simulink model "BFN_00_zfull_system"  (R2019b)
settings: Solver=VariableStepAuto  StartTime=0.0  StopTime=100  RelTol=1e-8
undefined symbols (not defined in the file): agh, Cd, dgh, Eearth, Esun, Gyro_freq, Gyro_noise_b, Gyro_noise_n, IFEHS_noise, Jsc, m_disturb, Magn_noise, q0, Surf_areas, Surf_dist, Surf_normals, Surf_reflectivity, targets_inertial, Tmax, today_mjd2000, w0
libraries: simulink x8, dspsrcs4 x2, vrlib x1
settings Model: Creator=Nicola  LastModifiedBy=Nicola

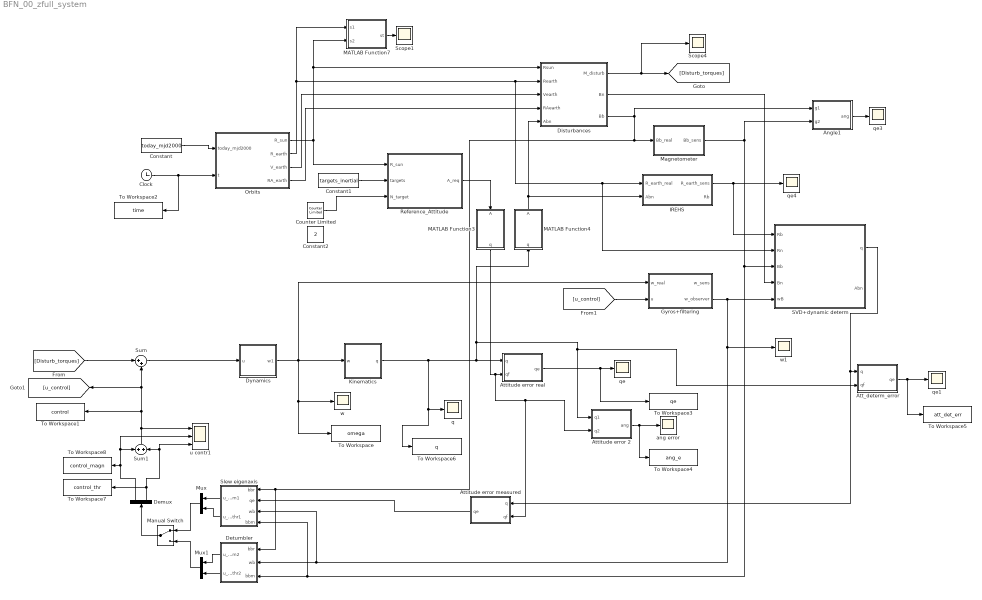
== system BFN_00_zfull_system ==
  Angle1 : MATLAB Function  TreatAsAtomicUnit=on
  Att_determ_error : MATLAB Function  TreatAsAtomicUnit=on
  Attitude error 2 : MATLAB Function  TreatAsAtomicUnit=on
  Attitude error measured : MATLAB Function  TreatAsAtomicUnit=on
  Attitude error real : MATLAB Function  TreatAsAtomicUnit=on
  Clock : Clock
  Constant : Constant  Value=today_mjd2000
  Constant1 : Constant  Value=targets_inertial
  Constant2 : Constant  Value=2
  Counter Limited : simulink/Sources/Counter Limited  uplimit=2  tsamp=6000*3
  Demux : Demux  Outputs=2
  Detumbler : Subsystem
  Disturbances : Subsystem
  Dynamics : Subsystem
  Gyros+filtering : Subsystem
  IREHS : Subsystem
  Kinematics : Subsystem
  MATLAB Function3 : MATLAB Function  TreatAsAtomicUnit=on
  MATLAB Function4 : MATLAB Function  TreatAsAtomicUnit=on
  MATLAB Function7 : MATLAB Function  TreatAsAtomicUnit=on
  Magnetometer : Subsystem
  Manual Switch : ManualSwitch
  Mux : Mux  Inputs=2
  Mux1 : Mux  Inputs=2
  Orbits : MATLAB Function  TreatAsAtomicUnit=on
  Reference_Attitude : MATLAB Function  TreatAsAtomicUnit=on
  SVD+dynamic determ : Subsystem
  Scope1 : Scope
  Scope4 : Scope
  Slew eigenaxis : Subsystem
  Sum : Sum  Inputs=|++
  Sum1 : Sum
  To Workspace : ToWorkspace  VariableName=omega  SampleTime=-1
      settings: Save2DSignal=2-D array (concatenate along first dimension)
  To Workspace1 : ToWorkspace  VariableName=control  SampleTime=-1
      settings: Save2DSignal=2-D array (concatenate along first dimension)
  To Workspace2 : ToWorkspace  VariableName=time  SampleTime=-1
      settings: Save2DSignal=2-D array (concatenate along first dimension)
  To Workspace3 : ToWorkspace  VariableName=qe  SampleTime=-1
      settings: Save2DSignal=2-D array (concatenate along first dimension)
  To Workspace4 : ToWorkspace  VariableName=ang_e  SampleTime=-1
      settings: Save2DSignal=2-D array (concatenate along first dimension)
  To Workspace5 : ToWorkspace  VariableName=att_det_err  SampleTime=-1
      settings: Save2DSignal=2-D array (concatenate along first dimension)
  To Workspace6 : ToWorkspace  VariableName=q  SampleTime=-1
      settings: Save2DSignal=2-D array (concatenate along first dimension)
  To Workspace7 : ToWorkspace  VariableName=control_thr  SampleTime=-1
      settings: Save2DSignal=2-D array (concatenate along first dimension)
  To Workspace8 : ToWorkspace  VariableName=control_magn  SampleTime=-1
      settings: Save2DSignal=2-D array (concatenate along first dimension)
  ang error : Scope
  q : Scope
  qe{,1,3..4} (4 alike) : Scope
  u contr1 : Scope  NumInputPorts=3
  w : Scope
  w1 : Scope
  wires:
  Constant/1 -> Orbits/1(today_mjd2000)
  Orbits/1(R_sun) -> Disturbances/1(Rsun), MATLAB Function7/2(s2), Reference_Attitude/1(R_sun)
  Constant1/1 -> Reference_Attitude/2(targets)
  Counter Limited/1 -> Reference_Attitude/3(N_target)
  Reference_Attitude/1(A_req) -> MATLAB Function3/1(A)
  Kinematics/1(q) -> To Workspace6/1, q/1, MATLAB Function4/1(q), Att_determ_error/2(qf), Attitude error 2/1(q1), Attitude error real/1(q)
  Attitude error real/1(qe) -> To Workspace3/1, qe/1
  MATLAB Function3/1(q) -> Attitude error measured/2(qf), Attitude error 2/2(q2), Attitude error real/2(qf)
  Sum/1 -> Dynamics/1(u)
  [Disturb_torques] -> Sum/1
  Disturbances/1(M_disturb) -> Scope4/1, [Disturb_torques]
  Orbits/2(R_earth) -> Disturbances/2(Rearth), IREHS/1(R_earth_real), SVD+dynamic determ/2(Rn), MATLAB Function7/1(s1)
  Orbits/3(V_earth) -> Disturbances/3(Vearth)
  Orbits/4(RA_earth) -> Disturbances/4(RAearth)
  MATLAB Function4/1(A) -> Disturbances/5(Abn), IREHS/2(Abn)
  [u_control] -> Gyros+filtering/2(u)
  Dynamics/1(w1) -> Gyros+filtering/1(w_real), w/1, To Workspace/1, Kinematics/1(w)
  Gyros+filtering/2(w_observer) -> Detumbler/2(wb), Slew eigenaxis/3(wb), w1/1, SVD+dynamic determ/5(wB)
  Disturbances/2(Bn) -> SVD+dynamic determ/4(Bn)
  IREHS/1(R_earth_sens) -> qe4/1, SVD+dynamic determ/1(Rb)
  Attitude error 2/1(ang) -> To Workspace4/1, ang error/1
  Disturbances/3(Bb) -> Detumbler/1(bbr), Slew eigenaxis/1(bbr), Magnetometer/1(Bb_real), Angle1/1(g1)
  Clock/1 -> To Workspace2/1, Orbits/2(t)
  SVD+dynamic determ/1(q) -> Attitude error measured/1(q), Att_determ_error/1(q)
  Magnetometer/1(Bb_sens) -> Angle1/2(g2), Detumbler/3(bbm), Slew eigenaxis/4(bbm), SVD+dynamic determ/3(Bb)
  Att_determ_error/1(qe) -> To Workspace5/1, qe1/1
  MATLAB Function7/1(st) -> Scope1/1
  Slew eigenaxis/1(u_contr_m1) -> Mux/1
  Attitude error measured/1(qe) -> Slew eigenaxis/2(qe)
  Angle1/1(ang) -> qe3/1
  Slew eigenaxis/2(u_contr_thr1) -> Mux/2
  Detumbler/2(u_contr_thr2) -> Mux1/2
  Detumbler/1(u_contr_m2) -> Mux1/1
  Mux/1 -> Manual Switch/1
  Mux1/1 -> Manual Switch/2
  Demux/1 -> To Workspace8/1, u contr1/2, Sum1/1
  Demux/2 -> To Workspace7/1, u contr1/3, Sum1/2
  Manual Switch/1 -> Demux/1
  Sum1/1 -> [u_control], Sum/2, To Workspace1/1, u contr1/1

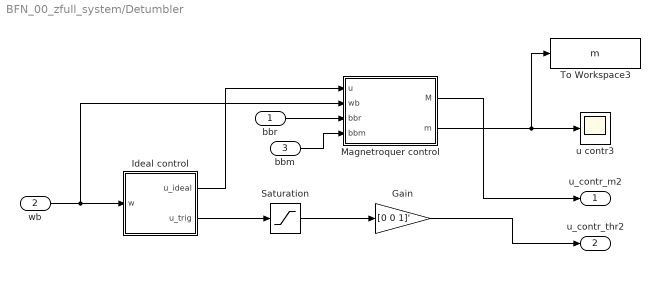
== system BFN_00_zfull_system/Detumbler ==
  bbr : Inport
  wb : Inport  Port=2
  bbm : Inport  Port=3
  Gain : Gain  Gain=[0 0 1]'
  Ideal control : Subsystem
  Magnetroquer control : MATLAB Function  TreatAsAtomicUnit=on
  Saturation : Saturate  UpperLimit=[1 1.7 1.7]'*2*Tmax  LowerLimit=[1 1.7 1.7]'*-2*Tmax
  To Workspace3 : ToWorkspace  VariableName=m  SampleTime=-1
      settings: Save2DSignal=2-D array (concatenate along first dimension)
  u contr3 : Scope
  u_contr_m2 : Outport
  u_contr_thr2 : Outport  Port=2
  wires:
  Magnetroquer control/1(M) -> u_contr_m2/1
  wb/1 -> Magnetroquer control/2(wb), Ideal control/1(w)
  Gain/1 -> u_contr_thr2/1
  Ideal control/1(u_ideal) -> Magnetroquer control/1(u)
  Magnetroquer control/2(m) -> To Workspace3/1, u contr3/1
  bbr/1 -> Magnetroquer control/3(bbr)
  Ideal control/2(u_trig) -> Saturation/1
  Saturation/1 -> Gain/1
  bbm/1 -> Magnetroquer control/4(bbm)

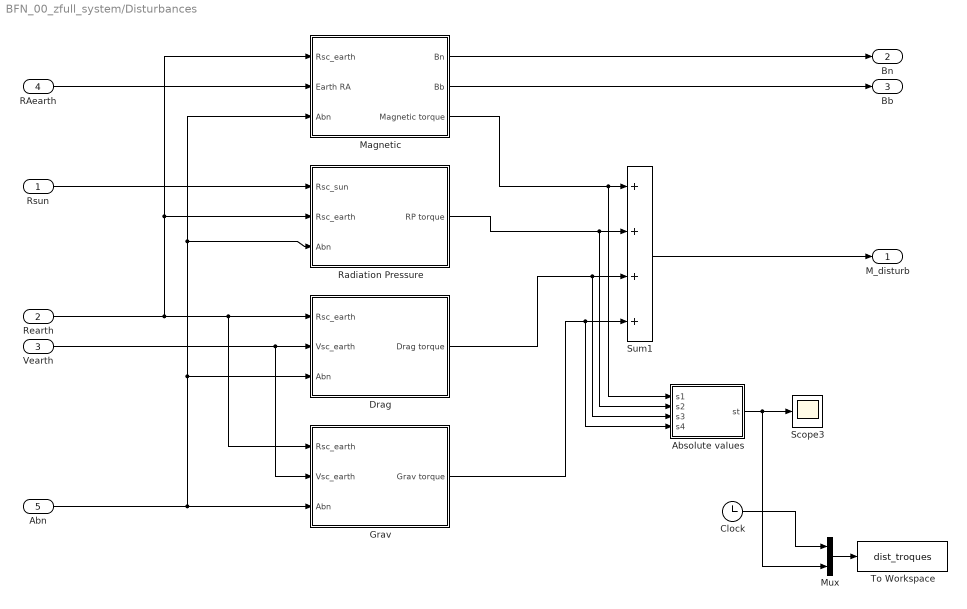
== system BFN_00_zfull_system/Disturbances ==
  Rsun : Inport
  Rearth : Inport  Port=2
  Vearth : Inport  Port=3
  RAearth : Inport  Port=4
  Abn : Inport  Port=5
  Absolute values : MATLAB Function  TreatAsAtomicUnit=on
  Clock : Clock
  Drag : Subsystem
  Grav : Subsystem
  Magnetic : Subsystem
  Mux : Mux  Inputs=2
  Radiation Pressure : Subsystem
  Scope3 : Scope
  Sum1 : Sum  Inputs=++++
  To Workspace : ToWorkspace  VariableName=dist_troques  SampleTime=-1
      settings: Save2DSignal=2-D array (concatenate along first dimension)
  M_disturb : Outport
  Bn : Outport  Port=2
  Bb : Outport  Port=3
  wires:
  Rsun/1 -> Radiation Pressure/1(Rsc_sun)
  Vearth/1 -> Grav/2(Vsc_earth), Drag/2(Vsc_earth)
  Abn/1 -> Magnetic/3(Abn), Radiation Pressure/3(Abn), Drag/3(Abn), Grav/3(Abn)
  Magnetic/3(Magnetic torque) -> Absolute values/1(s1), Sum1/1
  Absolute values/1(st) -> Mux/2, Scope3/1
  RAearth/1 -> Magnetic/2(Earth RA)
  Grav/1(Grav torque) -> Absolute values/4(s4), Sum1/4
  Rearth/1 -> Magnetic/1(Rsc_earth), Radiation Pressure/2(Rsc_earth), Grav/1(Rsc_earth), Drag/1(Rsc_earth)
  Radiation Pressure/1(RP torque) -> Absolute values/2(s2), Sum1/2
  Drag/1(Drag torque) -> Absolute values/3(s3), Sum1/3
  Sum1/1 -> M_disturb/1
  Magnetic/2(Bb) -> Bb/1
  Magnetic/1(Bn) -> Bn/1
  Clock/1 -> Mux/1
  Mux/1 -> To Workspace/1

== system BFN_00_zfull_system/Dynamics ==
  u : Inport
  I : Constant  Value=Jsc
  euler_eq : MATLAB Function  TreatAsAtomicUnit=on
  w : Integrator  InitialConditionSource=external
  w0 : Constant  Value=w0
  w1 : Outport
  wires:
  euler_eq/1(wd) -> w/1
  w0/1 -> w/2
  w/1 -> euler_eq/1(w), w1/1
  I/1 -> euler_eq/2(I)
  u/1 -> euler_eq/3(u)

== system BFN_00_zfull_system/Gyros+filtering ==
  w_real : Inport
  u : Inport  Port=2
  Gyro : Subsystem  Variant=on
  Scope1 : Scope
  w_sens : Outport
  w_observer : Outport  Port=2
  wires:
  w_real/1 -> Gyro/1(wr)
  u/1 -> Gyro/2(u)
  Gyro/2(w_observ) -> Scope1/1, w_observer/1
  Gyro/1(w_sens) -> w_sens/1

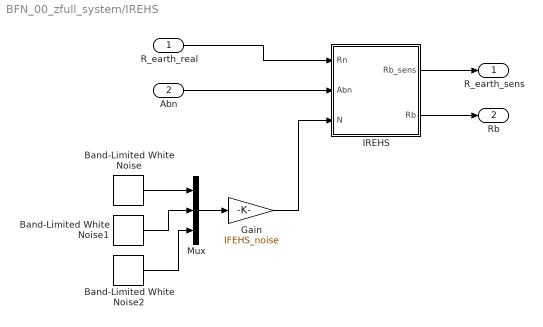
== system BFN_00_zfull_system/IREHS ==
  R_earth_real : Inport
  Abn : Inport  Port=2
  Band-Limited White Noise : simulink/Sources/Band-Limited White Noise  Cov=0.1  Ts=1  seed=[23341]
  Band-Limited White Noise1 : simulink/Sources/Band-Limited White Noise  Cov=0.1  Ts=1  seed=[598743]
  Band-Limited White Noise2 : simulink/Sources/Band-Limited White Noise  Cov=0.1  Ts=1  seed=[1235873]
  Gain : Gain  Gain=IFEHS_noise
  IREHS : MATLAB Function  TreatAsAtomicUnit=on
  Mux : Mux  Inputs=3
  R_earth_sens : Outport
  Rb : Outport  Port=2
  wires:
  R_earth_real/1 -> IREHS/1(Rn)
  Band-Limited White Noise/1 -> Mux/1
  Band-Limited White Noise1/1 -> Mux/2
  Band-Limited White Noise2/1 -> Mux/3
  Mux/1 -> Gain/1
  Abn/1 -> IREHS/2(Abn)
  IREHS/1(Rb_sens) -> R_earth_sens/1
  Gain/1 -> IREHS/3(N)
  IREHS/2(Rb) -> Rb/1

== system BFN_00_zfull_system/Kinematics ==
  w : Inport
  MATLAB Function : MATLAB Function  TreatAsAtomicUnit=on
  MATLAB Function5 : MATLAB Function  TreatAsAtomicUnit=on
  q0 : Constant  Value=q0
  quat : Integrator  InitialConditionSource=external
  q : Outport
  wires:
  quat/1 -> MATLAB Function5/1(q)
  q0/1 -> quat/2
  MATLAB Function/1(qd) -> quat/1
  w/1 -> MATLAB Function/2(w)
  MATLAB Function5/1(qn) -> MATLAB Function/1(q), q/1

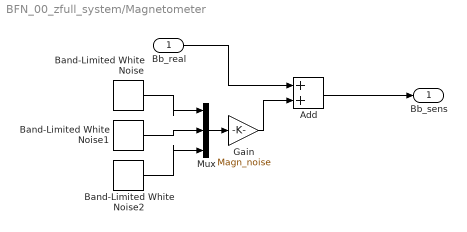
== system BFN_00_zfull_system/Magnetometer ==
  Bb_real : Inport
  Add : Sum
  Band-Limited White Noise : simulink/Sources/Band-Limited White Noise  Cov=0.1  Ts=1  seed=[23341]
  Band-Limited White Noise1 : simulink/Sources/Band-Limited White Noise  Cov=0.1  Ts=1  seed=[598743]
  Band-Limited White Noise2 : simulink/Sources/Band-Limited White Noise  Cov=0.1  Ts=1  seed=[1235873]
  Gain : Gain  Gain=Magn_noise
  Mux : Mux  Inputs=3
  Bb_sens : Outport
  wires:
  Add/1 -> Bb_sens/1
  Bb_real/1 -> Add/1
  Mux/1 -> Gain/1
  Band-Limited White Noise/1 -> Mux/1
  Band-Limited White Noise1/1 -> Mux/2
  Band-Limited White Noise2/1 -> Mux/3
  Gain/1 -> Add/2

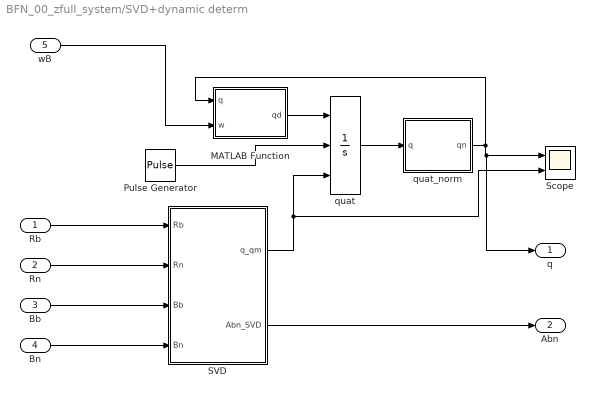
== system BFN_00_zfull_system/SVD+dynamic determ ==
  Rb : Inport
  Rn : Inport  Port=2
  Bb : Inport  Port=3
  Bn : Inport  Port=4
  wB : Inport  Port=5
  MATLAB Function : MATLAB Function  TreatAsAtomicUnit=on
  Pulse Generator : DiscretePulseGenerator  PulseType=Time based  Period=1  PulseWidth=5
  SVD : MATLAB Function  TreatAsAtomicUnit=on
  Scope : Scope  NumInputPorts=2
  quat : Integrator  ExternalReset=rising  InitialConditionSource=external
  quat_norm : MATLAB Function  TreatAsAtomicUnit=on
  q : Outport
  Abn : Outport  Port=2
  wires:
  quat_norm/1(qn) -> q/1, Scope/1, MATLAB Function/1(q)
  MATLAB Function/1(qd) -> quat/1
  quat/1 -> quat_norm/1(q)
  wB/1 -> MATLAB Function/2(w)
  Pulse Generator/1 -> quat/2
  Bn/1 -> SVD/4(Bn)
  Bb/1 -> SVD/3(Bb)
  Rn/1 -> SVD/2(Rn)
  Rb/1 -> SVD/1(Rb)
  SVD/2(Abn_SVD) -> Abn/1
  SVD/1(q_qm) -> Scope/2, quat/3

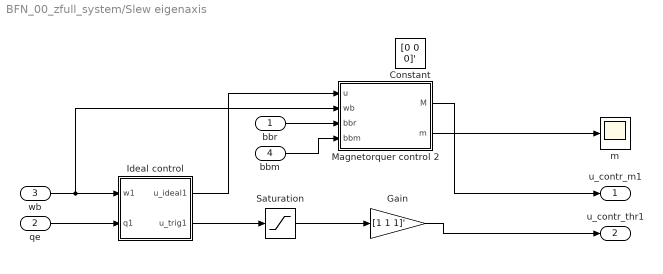
== system BFN_00_zfull_system/Slew eigenaxis ==
  bbr : Inport
  qe : Inport  Port=2
  wb : Inport  Port=3
  bbm : Inport  Port=4
  Constant : Constant  Value=[0 0 0]'
  Gain : Gain  Gain=[1 1 1]'
  Ideal control : Subsystem
  Magnetorquer control 2 : MATLAB Function  TreatAsAtomicUnit=on
  Saturation : Saturate  UpperLimit=[1 1.7 1.7]'*2*Tmax  LowerLimit=[1 1.7 1.7]'*-2*Tmax
  m : Scope
  u_contr_m1 : Outport
  u_contr_thr1 : Outport  Port=2
  wires:
  wb/1 -> Magnetorquer control 2/2(wb), Ideal control/1(w1)
  Ideal control/1(u_ideal1) -> Magnetorquer control 2/1(u)
  Magnetorquer control 2/1(M) -> u_contr_m1/1
  Magnetorquer control 2/2(m) -> m/1
  bbr/1 -> Magnetorquer control 2/3(bbr)
  qe/1 -> Ideal control/2(q1)
  bbm/1 -> Magnetorquer control 2/4(bbm)
  Ideal control/2(u_trig1) -> Saturation/1
  Gain/1 -> u_contr_thr1/1
  Saturation/1 -> Gain/1

== system BFN_00_zfull_system/Detumbler/Ideal control ==
  w : Inport
  Detumbl : MATLAB Function  TreatAsAtomicUnit=on
  Memory : Memory  InitialCondition=[0 0 0]'
  u_ideal : Outport
  u_trig : Outport  Port=2
  wires:
  Detumbl/1(u_trig) -> u_trig/1
  w/1 -> Detumbl/1(w)
  Detumbl/3(H) -> Memory/1
  Memory/1 -> Detumbl/2("H ")
  Detumbl/2(u) -> u_ideal/1

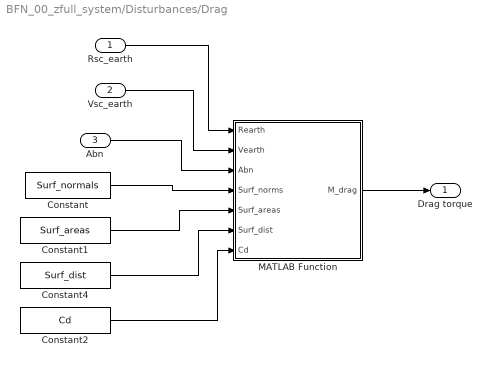
== system BFN_00_zfull_system/Disturbances/Drag ==
  Rsc_earth : Inport
  Vsc_earth : Inport  Port=2
  Abn : Inport  Port=3
  Constant : Constant  Value=Surf_normals
  Constant1 : Constant  Value=Surf_areas
  Constant2 : Constant  Value=Cd
  Constant4 : Constant  Value=Surf_dist
  MATLAB Function : MATLAB Function  TreatAsAtomicUnit=on
  Drag torque : Outport
  wires:
  Abn/1 -> MATLAB Function/3(Abn)
  Rsc_earth/1 -> MATLAB Function/1(Rearth)
  MATLAB Function/1(M_drag) -> Drag torque/1
  Constant/1 -> MATLAB Function/4(Surf_norms)
  Constant1/1 -> MATLAB Function/5(Surf_areas)
  Constant4/1 -> MATLAB Function/6(Surf_dist)
  Vsc_earth/1 -> MATLAB Function/2(Vearth)
  Constant2/1 -> MATLAB Function/7(Cd)

== system BFN_00_zfull_system/Disturbances/Grav ==
  Rsc_earth : Inport
  Vsc_earth : Inport  Port=2
  Abn : Inport  Port=3
  Constant : Constant  Value=Jsc
  MATLAB Function : MATLAB Function  TreatAsAtomicUnit=on
  Grav torque : Outport
  wires:
  Abn/1 -> MATLAB Function/3(Abn)
  Rsc_earth/1 -> MATLAB Function/1(Rearth)
  MATLAB Function/1(M_grav) -> Grav torque/1
  Constant/1 -> MATLAB Function/4(J)
  Vsc_earth/1 -> MATLAB Function/2(Vearth)

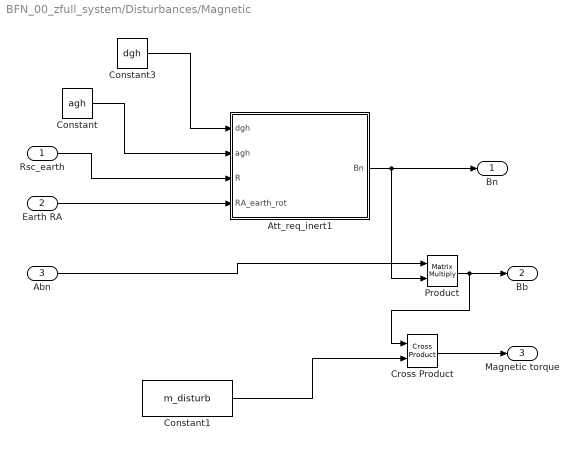
== system BFN_00_zfull_system/Disturbances/Magnetic ==
  Rsc_earth : Inport
  Earth RA : Inport  Port=2
  Abn : Inport  Port=3
  Att_req_inert1 : MATLAB Function  TreatAsAtomicUnit=on
  Constant : Constant  Value=agh
  Constant1 : Constant  Value=m_disturb
  Constant3 : Constant  Value=dgh
  Cross Product : vrlib/Utilities/Cross Product
      settings: SourceProductName=Simulink
  Product : Product  Multiplication=Matrix(*)
  Bn : Outport
  Bb : Outport  Port=2
  Magnetic torque : Outport  Port=3
  wires:
  Att_req_inert1/1(Bn) -> Product/2, Bn/1
  Rsc_earth/1 -> Att_req_inert1/3(R)
  Constant3/1 -> Att_req_inert1/1(dgh)
  Constant/1 -> Att_req_inert1/2(agh)
  Earth RA/1 -> Att_req_inert1/4(RA_earth_rot)
  Abn/1 -> Product/1
  Product/1 -> Cross Product/1, Bb/1
  Constant1/1 -> Cross Product/2
  Cross Product/1 -> Magnetic torque/1

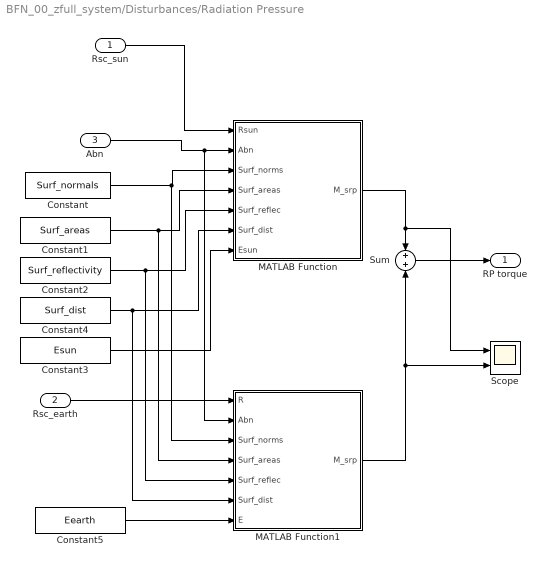
== system BFN_00_zfull_system/Disturbances/Radiation Pressure ==
  Rsc_sun : Inport
  Rsc_earth : Inport  Port=2
  Abn : Inport  Port=3
  Constant : Constant  Value=Surf_normals
  Constant1 : Constant  Value=Surf_areas
  Constant2 : Constant  Value=Surf_reflectivity
  Constant3 : Constant  Value=Esun
  Constant4 : Constant  Value=Surf_dist
  Constant5 : Constant  Value=Eearth
  MATLAB Function : MATLAB Function  TreatAsAtomicUnit=on
  MATLAB Function1 : MATLAB Function  TreatAsAtomicUnit=on
  Scope : Scope  NumInputPorts=2
  Sum : Sum
  RP torque : Outport
  wires:
  Abn/1 -> MATLAB Function1/2(Abn), MATLAB Function/2(Abn)
  Rsc_sun/1 -> MATLAB Function/1(Rsun)
  MATLAB Function/1(M_srp) -> Scope/1, Sum/1
  Constant/1 -> MATLAB Function1/3(Surf_norms), MATLAB Function/3(Surf_norms)
  Constant1/1 -> MATLAB Function1/4(Surf_areas), MATLAB Function/4(Surf_areas)
  Constant2/1 -> MATLAB Function1/5(Surf_reflec), MATLAB Function/5(Surf_reflec)
  Constant3/1 -> MATLAB Function/7(Esun)
  Constant4/1 -> MATLAB Function1/6(Surf_dist), MATLAB Function/6(Surf_dist)
  Sum/1 -> RP torque/1
  MATLAB Function1/1(M_srp) -> Sum/2, Scope/2
  Rsc_earth/1 -> MATLAB Function1/1(R)
  Constant5/1 -> MATLAB Function1/7(E)

== system BFN_00_zfull_system/Gyros+filtering/Gyro ==
  note: 1) Add Subsystem or Model blocks as valid variant choices.
      | 2) You cannot connect blocks at this level. At simulation, connectivity is automatically
      | determined, based on the active variant and port name matching.
  wr : Inport
  u : Inport  Port=2
  Gyro+observer : Subsystem  VariantControl=Gyro_Bypass_1
  bypass : Subsystem  VariantControl=Gyro_Bypass_2
  w_sens : Outport
  w_observ : Outport  Port=2

== system BFN_00_zfull_system/Slew eigenaxis/Ideal control ==
  w1 : Inport
  q1 : Inport  Port=2
  Constant : Constant  Value=Jsc
  Memory : Memory  InitialCondition=[0 0 0]'
  eigenaxis slew : MATLAB Function  TreatAsAtomicUnit=on
  u_ideal1 : Outport
  u_trig1 : Outport  Port=2
  wires:
  eigenaxis slew/1(u_trig) -> u_trig1/1
  w1/1 -> eigenaxis slew/1(w)
  q1/1 -> eigenaxis slew/2(qe)
  Constant/1 -> eigenaxis slew/3(I)
  eigenaxis slew/3(H) -> Memory/1
  Memory/1 -> eigenaxis slew/4("H ")
  eigenaxis slew/2(u) -> u_ideal1/1

== system BFN_00_zfull_system/Gyros+filtering/Gyro/Gyro+observer ==
  wr : Inport
  u : Inport  Port=2
  3d_gyro : Subsystem
  observer : Subsystem
  w_sens : Outport
  w_observ : Outport  Port=2
  wires:
  u/1 -> observer/2(u)
  3d_gyro/1(w_sens) -> w_sens/1, observer/1(w)
  wr/1 -> 3d_gyro/1(w)
  observer/1(w_obs) -> w_observ/1

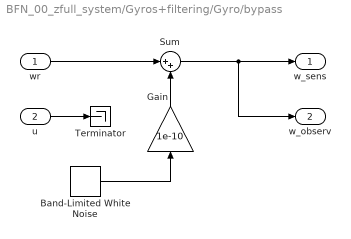
== system BFN_00_zfull_system/Gyros+filtering/Gyro/bypass ==
  wr : Inport
  u : Inport  Port=2
  Band-Limited White Noise : simulink/Sources/Band-Limited White Noise  Cov=[0.1]  Ts=0.5  seed=[23341]
  Gain : Gain  Gain=1e-10
  Sum : Sum  Inputs=|++
  Terminator : Terminator
  w_sens : Outport
  w_observ : Outport  Port=2
  wires:
  Sum/1 -> w_observ/1, w_sens/1
  u/1 -> Terminator/1
  wr/1 -> Sum/1
  Band-Limited White Noise/1 -> Gain/1
  Gain/1 -> Sum/2

== system BFN_00_zfull_system/Gyros+filtering/Gyro/Gyro+observer/3d_gyro ==
  w : Inport
  Gain : Gain  Gain=1e5
  Integrator2 : Integrator  InitialCondition=[0 0 0]'
  Noise : Subsystem
  Scope1 : Scope  NumInputPorts=2
  Sum : Sum  Inputs=|+-
  Sum1 : Sum  Inputs=||+++
  w_sens : Outport
  wires:
  Integrator2/1 -> Sum/2, Sum1/1
  Noise/2(b) -> Scope1/2, Sum1/3
  Sum1/1 -> w_sens/1
  Noise/1(n) -> Scope1/1, Sum1/2
  Sum/1 -> Gain/1
  w/1 -> Sum/1
  Gain/1 -> Integrator2/1

== system BFN_00_zfull_system/Gyros+filtering/Gyro/Gyro+observer/observer ==
  w : Inport
  u : Inport  Port=2
  I : Constant  Value=Jsc
  Integrator : Integrator  InitialCondition=[0.42 0.52 0.55 ]'
  MATLAB Function : MATLAB Function  TreatAsAtomicUnit=on
  w_obs : Outport
  wires:
  Integrator/1 -> MATLAB Function/1(w), w_obs/1
  MATLAB Function/1(w_obs_d) -> Integrator/1
  u/1 -> MATLAB Function/4(u)
  w/1 -> MATLAB Function/2(w_sens)
  I/1 -> MATLAB Function/3(I)

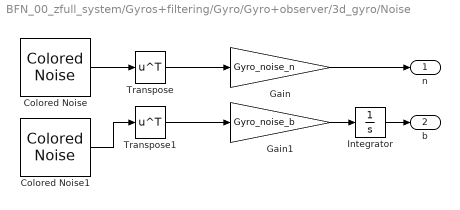
== system BFN_00_zfull_system/Gyros+filtering/Gyro/Gyro+observer/3d_gyro/Noise ==
  Colored Noise : dspsrcs4/Colored Noise  Color=white  InverseFrequencyPower=1  BoundedOutput=off  NumChannels=3  OutputDataType=double  SamplesPerFrame=1  SampleTime=1/Gyro_freq  RandomStream=mt19937ar with seed  Seed=67  SimulateUsing=Interpreted execution
      settings: SourceProductName=DSP System Toolbox  SourceProductBaseCode=DS
  Colored Noise1 : dspsrcs4/Colored Noise  Color=white  InverseFrequencyPower=1  BoundedOutput=off  NumChannels=3  OutputDataType=double  SamplesPerFrame=1  SampleTime=1/Gyro_freq  RandomStream=mt19937ar with seed  Seed=34  SimulateUsing=Interpreted execution
      settings: SourceProductName=DSP System Toolbox  SourceProductBaseCode=DS
  Gain : Gain  Gain=Gyro_noise_n
  Gain1 : Gain  Gain=Gyro_noise_b
  Integrator : Integrator  InitialCondition=[3 -3 0]'*Gyro_noise_b*1e-2*0
  Transpose : Math  Operator=transpose  SignedPower=off  SaturateOnIntegerOverflow=on
  Transpose1 : Math  Operator=transpose  SignedPower=off  SaturateOnIntegerOverflow=on
  n : Outport
  b : Outport  Port=2
  wires:
  Transpose/1 -> Gain/1
  Integrator/1 -> b/1
  Colored Noise/1 -> Transpose/1
  Gain1/1 -> Integrator/1
  Gain/1 -> n/1
  Transpose1/1 -> Gain1/1
  Colored Noise1/1 -> Transpose1/1

== matlab function BFN_00_zfull_system/Disturbances/Radiation Pressure/MATLAB Function ==
  data: Rsun input; M_srp output; Abn input; Surf_norms input; Surf_areas input; Surf_reflec input; Surf_dist input; Esun input
function M_srp = SRP(Rsun,Abn,Surf_norms,Surf_areas,Surf_reflec,Surf_dist,Esun)
%SRP finds torque due to SRP
Sb = Abn*(-Rsun/norm(Rsun));
c = 299792458;%[m/s] speed of light
P = Esun/c;%[Pa] Pressure
tmp1=ones(3,6);
tmp2=dot(bsxfun(@times, tmp1,Sb),Surf_norms);

% F = -P*Surf_areas'.*tmp2.*((1-Surf_reflec').*Sb+...
%     (2*Surf_reflec'.*tmp2+2/3*Surf_reflec').*Surf_normals);

one = -P*bsxfun(@times,Surf_areas',tmp2);
two = bsxfun(@times,(1-Surf_reflec'),Sb);
three = 2*bsxfun(@times,Surf_reflec',tmp2);
four = bsxfun(@times,(three+2/3*Surf_reflec'),Surf_norms);
F = bsxfun(@times,one,(two+four));%[N] forces acting
M_srp = sum(bsxfun(@times,cross(Surf_dist,F),(tmp2>0)),2);%[Nm] Torque

== matlab function BFN_00_zfull_system/Orbits ==
  data: today_mjd2000 input; t input; R_sun output; R_earth output; V_earth output; RA_earth output
function [R_sun,R_earth,V_earth,RA_earth] = orbit_determ(today_mjd2000,t)
%ORBIT_DETERM calculates earth and sc position with time
%   INPUT mjd2000 date, time in seconds
%   OUTPUT sc position in sun inertial, position in earth inertial
%          sc velocity in ECI, earth siderial time.
M0 = 1.8832;%[rad] initial Mean Anomaly
Mue = 398600.4418;%[km3/s2)]Earth gravity parameter
ecliptic = (23+26/60+21.4119/3600)*pi/180;%[rad]
%Dates calc
now_mjd2000 = today_mjd2000 + t/86400;%[days] mjd2000

%Earth in equatorial heliocentric inertial in m
[Earth_kep1, Mus] = uplanet (now_mjd2000, 3);
[R_Earth, ~] = kep2car_v1(Earth_kep1, Mus);
R_Earth = (rot('x',-ecliptic)*R_Earth')*1e3;%[km]
%Spacecraft equatorial geocentric inertial
a = (800+6375);%km semimajor axis
e = 1e-3;%eccentricity
i = 45*pi/180;%[rad] inclination
RA = 33*pi/180;%[rad] right accention
n = sqrt(Mue/a^3);%[rad/s] mean motion
M = n*t+M0;%[rad] mean anomaly
TA = MA2TA(M,e);%[rad] true anomaly
%[a e RA incl w TA]
kep_sc = [a e RA i 0 TA];% kepler elements
[R_earth1, V_earth1] = kep2car_v1(kep_sc,Mue);
R_earth=R_earth1'*1e3; V_earth= V_earth1'*1e3;
R_sun = R_Earth + R_earth;
n_earth_rot = 1/86164.098903691;%Hz
RA_earth = n_earth_rot*t+now_mjd2000/365;%Earth RA or siderial time
RA_earth = 2*pi*(RA_earth-fix(RA_earth));

== matlab function BFN_00_zfull_system/Reference_Attitude ==
  data: R_sun input; targets input; A_req output; N_target input
function A_req = ref_attitude(R_sun,targets,N_target)
%REF_ATTITUDE calculates reference attiture pointing X to target, Y to sun
R_sun = R_sun/norm(R_sun);

%Ref attitude creation
A = [targets(:,N_target+1) R_sun cross(targets(:,N_target+1),R_sun)];
% matrix orthonormalization
for i=1:5
    A = A*3/2-A*(A')*A/2;
end
A_req = A;

== matlab function BFN_00_zfull_system/Dynamics/euler_eq ==
  data: w input; wd output; I input; u input
function wd = euler_eq(w,I,u)
%EULER equation
J=diag(I);
wd = J\(cross(J*w,w)+u);

== matlab function BFN_00_zfull_system/Kinematics/MATLAB Function ==
  data: q input; qd output; w input
function qd = quat(q,w)
%Kinematics
qd = hat4(w)*q/2;

== matlab function BFN_00_zfull_system/Attitude error real ==
  data: q input; qe output; qf input
function qe = quat_error(q,qf)
%Calc Attitude error between reference and actual attitudes
qe = hat4q(qf)*q;

== matlab function BFN_00_zfull_system/Kinematics/MATLAB Function5 ==
  data: q input; qn output
function qn = normalize(q)
%quaternion normalization
qn = q/sqrt(sum(q.^2));

== matlab function BFN_00_zfull_system/Slew eigenaxis/Magnetorquer control 2 ==
  data: u input; wb input; M output; bbr input; m output; bbm input
function [M,m]  = magnetorquer(u,wb,bbr,bbm)
%calcs m for mognetorquer control
n=2;
switch n
    case 1
        m=-1e7*cross(bbm,wb);
    case 2
        m = 1e-1*cross(bbm,u)/dot(bbm,bbm);
    case 3
        m = 1/bbm(3)*[0 -1 0;1 0 0;bbm']*u/10;
end
m=saturation(m,1.5);
M=cross(m,bbr);

== matlab function BFN_00_zfull_system/MATLAB Function3 ==
  data: A input; q output
function q = A2q1(A)
% DCN to quaternion
q = A2q(A);

== matlab function BFN_00_zfull_system/Disturbances/Magnetic/Att_req_inert1 ==
  data: dgh input; agh input; R input; Bn output; RA_earth_rot input
function Bn = magn_field(dgh,agh,R,RA_earth_rot)
%MAGN_FIELD finds magnetic field values using IGRF13 model
Sphc = car2spher(R);
%[Right accencion [rad], declination [rad], radius [whatever]]
Sphc(1) = Sphc(1)-RA_earth_rot;
B1 = magfd(2020,2,Sphc(3)/1000,Sphc(2),Sphc(1),dgh,agh).*[-1 1 -1]';
%B[colat,azimut,radial]
Bn = [(B1(3)*cos(Sphc(2))+B1(1)*sin(Sphc(2)))*cos(Sphc(1))-B1(2)*sin(Sphc(1));...
    (B1(3)*cos(Sphc(2))+B1(1)*sin(Sphc(2)))*sin(Sphc(1))+B1(2)*cos(Sphc(1));...
    B1(3)*sin(Sphc(2))-B1(1)*cos(Sphc(2))];

== matlab function BFN_00_zfull_system/MATLAB Function4 ==
  data: q input; A output
function A = q2A1(q)
%quaternion to DCN
A = q2A(q);

== matlab function BFN_00_zfull_system/Disturbances/Drag/MATLAB Function ==
  data: Rearth input; Vearth input; M_drag output; Abn input; Surf_norms input; Surf_areas input; Surf_dist input; Cd input
function M_drag = Drag_torque(Rearth,Vearth,Abn,Surf_norms,Surf_areas,Surf_dist,Cd)
%DRAG_TORQUE finds torque due to aerodynamic drag
w_earth = [0 0 0.000072921]';%[rad/s] earth rotation
v_rel = Vearth-cross(w_earth,Rearth);%[m/s] relative velocity
dens = 3.614e-14*exp(-((norm(Rearth)*1e-3-6375)-700)/88.667);%[kg/m3] interpolation
vrb = Abn*v_rel;
vrbabs = norm(vrb);
vrbv = vrb/vrbabs;
tmp1 = ones(3,6);
tmp2 = dot(Surf_norms,bsxfun(@times, tmp1,vrbv));
Across = Surf_areas'.*tmp2;
F = -1/2*dens*Cd*vrbabs^2*bsxfun(@times,vrbv,Across);%[N]
tmp3 = bsxfun(@times,[1 1 1]',tmp2>0);
M_drag = -sum(cross(Surf_dist,F).*tmp3,2);%[Nm]

== matlab function BFN_00_zfull_system/Disturbances/Radiation Pressure/MATLAB Function1 ==
  data: R input; M_srp output; Abn input; Surf_norms input; Surf_areas input; Surf_reflec input; Surf_dist input; E input
function M_srp = Albedo(R,Abn,Surf_norms,Surf_areas,Surf_reflec,Surf_dist,E)
%ALBEDO finds torque doe to Earth albedo radiation pressure
Sb = Abn*(-R/norm(R));
c = 299792458;%speed of light m/s
P = E/c;
tmp1=ones(3,6);
tmp2=dot(bsxfun(@times, tmp1,Sb),Surf_norms);

% F = -P*Surf_areas'.*tmp2.*((1-Surf_reflec').*Sb+...
%     (2*Surf_reflec'.*tmp2+2/3*Surf_reflec').*Surf_normals);

one = -P*bsxfun(@times,Surf_areas',tmp2);
two = bsxfun(@times,(1-Surf_reflec'),Sb);
three = 2*bsxfun(@times,Surf_reflec',tmp2);
four = bsxfun(@times,(three+2/3*Surf_reflec'),Surf_norms);
F = bsxfun(@times,one,(two+four));
%M_srp=[0 0 0]';
M_srp = sum(bsxfun(@times,cross(Surf_dist,F),(tmp2>0)),2);

== matlab function BFN_00_zfull_system/Disturbances/Grav/MATLAB Function ==
  data: Rearth input; Vearth input; Abn input; J input; M_grav output
function M_grav = Grav(Rearth,Vearth,Abn,J)
%GRAV calculates torque due to gravity
Mue = 398600.4418e3;%[km3/s2)]Earth gravity parameter
R1 = Rearth/norm(Rearth);
V1 = Vearth/norm(Vearth);
Aln = [R1 V1 cross(R1,V1)];
Abl = Abn/Aln;

M_grav = 3*Mue/norm(Rearth)^3*[(J(3)-J(2))*Abl(3,1)*Abl(2,1);...
                            (J(1)-J(3))*Abl(1,1)*Abl(3,1);...
                            (J(2)-J(1))*Abl(1,1)*Abl(2,1)];

== matlab function BFN_00_zfull_system/Disturbances/Absolute values ==
  data: s1 input; st output; s2 input; s3 input; s4 input
function st = absolutes(s1,s2,s3,s4)
%calculate absolute disurbance values
st = sqrt(sum([s1 s2 s3 s4].^2,1));

== matlab function BFN_00_zfull_system/IREHS/IREHS ==
  data: Rn input; Rb_sens output; Abn input; N input; Rb output
function [Rb_sens, Rb] = IREHS(Rn,Abn,N)
%IREHS calculates earth in body frame
Rn = Rn/norm(Rn);
Rb = Abn*Rn;
Rb_sens = Rb+N;
Rb_sens = Rb_sens/norm(Rb_sens);

== matlab function BFN_00_zfull_system/SVD+dynamic determ/SVD ==
  data: Rb input; q_qm output; Rn input; Bb input; Bn input; Abn_SVD output
function [q_qm,Abn_SVD] = SVD(Rb,Rn,Bb,Bn)
%SVD single value decomposition attitude determination
Rb=Rb/norm(Rb);
Rn=Rn/norm(Rn);
Bb=Bb/norm(Bb);
Bn=Bn/norm(Bn);
alph = [1 1];
alph = alph/norm(alph);
B = B_calc([Rb Bb],[Rn Bn],alph);
[U, ~, V] = svd(B);
Abn_SVD = U*diag([1 1 det(U)*det(V)])*V';
q_qm = A2q(Abn_SVD);

== matlab function BFN_00_zfull_system/Attitude error 2 ==
  data: q1 input; ang output; q2 input
function ang = angle(q1,q2)
%Calcs attitude error in terms of an angle between pointiong vectors
th1 = sqrt(1-q1(4)^2);
th2 = sqrt(1-q2(4)^2);
g1 = q1(1:3)/th1;
g2 = q2(1:3)/th2;
ang = acos(dot(g1,g2)/norm(g1)/norm(g2))*180/pi;
if ang>90
    ang=ang-180; 
end

== matlab function BFN_00_zfull_system/Gyros+filtering/Gyro/Gyro+observer/observer/MATLAB Function ==
  data: w input; w_sens input; I input; u input; w_obs_d output
function w_obs_d = observer(w,w_sens,I,u)
%OBSERVER low pass filter
al = -0.5;
J=diag(I);
w_obs_d = J\(cross(J*w,w)+u+al*(w-w_sens));

== matlab function BFN_00_zfull_system/SVD+dynamic determ/MATLAB Function ==
  data: q input; qd output; w input
function qd = quat(q,w)
%QUAT calculates q_dot given angular velocities
qd = hat4(w)*q/2;

== matlab function BFN_00_zfull_system/SVD+dynamic determ/quat_norm ==
  data: q input; qn output
function qn = normalize(q)
%quaternion normialization
qn = q/sqrt(sum(q.^2));

== matlab function BFN_00_zfull_system/Att_determ_error ==
  data: q input; qe output; qf input
function qe = quat_error(q,qf)
%Calcl attitude determination error
qe = hat4q(qf)*q;

== matlab function BFN_00_zfull_system/Slew eigenaxis/Ideal control/eigenaxis slew ==
  data: u_trig output; w input; qe input; u output; I input; H input; H output
function [u_trig,u,H]  = q_contr1(w,qe,I,H)
%Slew eigenaxis control law
k1=1;
k2=k1^2/2;
n=4;
switch n
    case 1
        dhdq = @(q)-1;
    case 2
        dhdq = @(q)1;
    case 3
        dhdq = @(q)-2*q;
    case 4
        dhdq = @(q)-1/q;
    case 5
        dhdq = @(q)-2*acos(q)/sqrt(1-q^2);
    otherwise
        dhdq = @(q)-1;
end
J=diag(I);
u = k1*(J*-w+saturation(cross(w,J*w)/k1+k2/k1*dhdq(qe(4))*J*qe(1:3),0.0005));%0.0005
%Shmitd trigger
uplim = 1e-5;
downlim = 3e-8;
H = [1 1 1]'.*(sum([abs(u)>uplim abs(u)>downlim H],2)>1);
u_trig = u.*H;

== matlab function BFN_00_zfull_system/MATLAB Function7 ==
  data: s1 input; st output; s2 input
function st = absolutes(s1,s2)
st = sqrt(sum([s1 s2].^2,1));

== matlab function BFN_00_zfull_system/Detumbler/Magnetroquer control ==
  data: u input; wb input; M output; bbr input; m output; bbm input
function [M,m]  = magnetorquer(u,wb,bbr,bbm)
%Calcs magnetorquer m control for detumbling
n=1;
switch n
    case 1
        m=-1e7*cross(bbm,wb);
    case 2
        m = 1e-1*cross(bbm,u)/dot(bbm,bbm);
    case 3
        m = 1/bbm(3)*[0 -1 0;1 0 0;bbm']*u/10;
end
m=saturation(m,1.5);
M=cross(m,bbr);

== matlab function BFN_00_zfull_system/Detumbler/Ideal control/Detumbl ==
  data: u_trig output; w input; u output; H input; H output
function [u_trig,u,H]  = detumbler(w,H)
k=0.5;
u=-k*w;
%shmidt trigger
uplim = 3e-5;
downlim = 1e-6;
H = [1 1 1]'.*(sum([abs(u)>uplim abs(u)>downlim H],2)>1);
u_trig = u.*H;

== matlab function BFN_00_zfull_system/Attitude error measured ==
  data: q input; qe output; qf input
function qe = quat_error(q,qf)
%Calc Attitude error based on sensor data
qe = hat4q(qf)*q;

== matlab function BFN_00_zfull_system/Angle1 ==
  data: g1 input; ang output; g2 input
function ang = angle(g1,g2)
%ANGLE calc angle between 2 vectors
ang = acos(dot(g1,g2)/norm(g1)/norm(g2))*180/pi;
if ang>90
    ang=ang-180; 
end
